simulink model "Modulator_CTDT"  (R2025b)
settings: Solver=ode4  StartTime=0.0  StopTime=0.5  FixedStep=Ts/10  MaxStep=1e-6  RelTol=1e-3
values from neighbouring files (symbols this model uses):
  Fs = 512e3    (= 512000)    [initialize_parameters_CTDT.m]
  Ts = 1/Fs    (= 1.953125e-06)    [initialize_parameters_CTDT.m]
undefined symbols (not defined in the file or in its folder): den, dspblkCoreblockFVToolHelper, gcbh, num
libraries: dspmlti4 x1
settings Model: Creator=anurag jaiswal  LastModifiedBy=divijsharma
settings DataIOCC: SaveOutput=off  SignalLogging=off  DSMLogging=off  SaveTime=off  ReturnWorkspaceOutputs=off

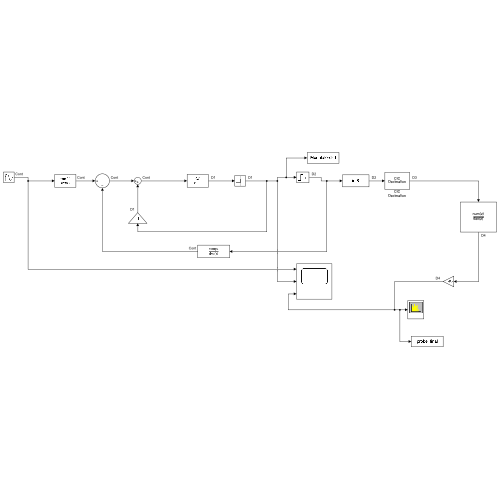
[thumbnail: Simulink's stored preview of the top-level diagram]
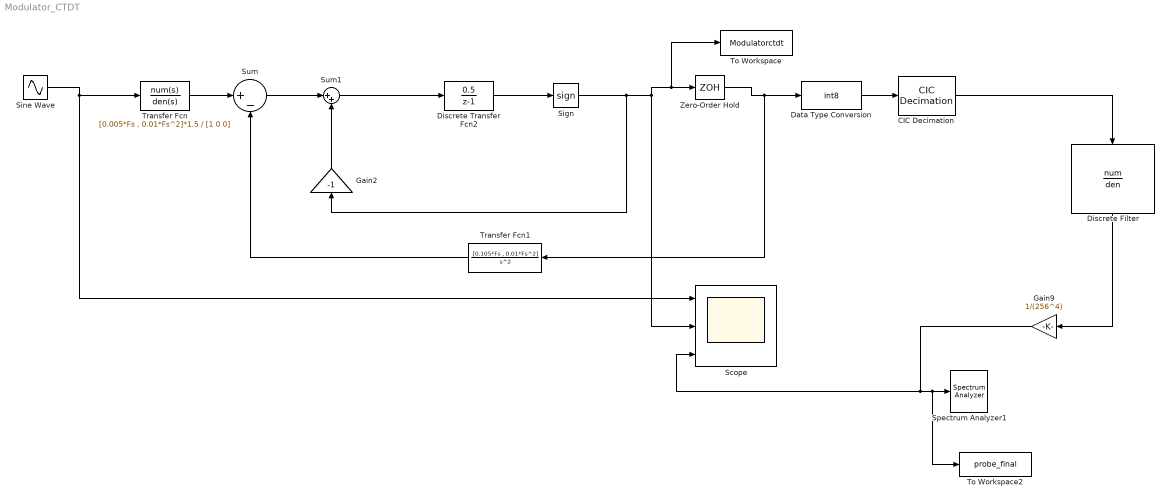
== system Modulator_CTDT ==
  CIC Decimation : dspmlti4/CIC Decimation  filtFrom=Dialog parameters  filtobj=CICDECIM  ftype=Decimator  R=256  M=1  N=5  filterInternals=Minimum section word lengths  BPS=[16 16 16 16]  FLPS=0  outputWordLength=32  outputFracLength=0  launchFVT=off  framing=Maintain input frame rate  RateOptions=Allow multirate processing
      settings: LibrarySourceBlock=|
      | dsphdlsupportfiltering/CIC
      | Decimation
  Data Type Conversion : DataTypeConversion  OutDataTypeStr=int8  SaturateOnIntegerOverflow=off  RndMeth=Floor
  Discrete Transfer Fcn2 : DiscreteTransferFcn  LoadFcn=dspblkCoreblockFVToolHelper(gcbh,'load');  Numerator=[0.5]  Denominator=[1 -1]
      settings: CopyFcn=dspblkCoreblockFVToolHelper(gcbh,'copy');  DeleteFcn=dspblkCoreblockFVToolHelper(gcbh,'close');  ModelCloseFcn=dspblkCoreblockFVToolHelper(gcbh,'close');  PreSaveFcn=dspblkCoreblockFVToolHelper(gcbh,'presave');  PostSaveFcn=dspblkCoreblockFVToolHelper(gcbh,'postsave');  CloseFcn=dspblkCoreblockFVToolHelper(gcbh,'close');
  Discrete Filter : DiscreteFilter  LoadFcn=dspblkCoreblockFVToolHelper(gcbh,'load');  Numerator=num  Denominator=den
      settings: CopyFcn=dspblkCoreblockFVToolHelper(gcbh,'copy');  DeleteFcn=dspblkCoreblockFVToolHelper(gcbh,'close');  ModelCloseFcn=dspblkCoreblockFVToolHelper(gcbh,'close');  PreSaveFcn=dspblkCoreblockFVToolHelper(gcbh,'presave');  PostSaveFcn=dspblkCoreblockFVToolHelper(gcbh,'postsave');  CloseFcn=dspblkCoreblockFVToolHelper(gcbh,'close');
  Gain2 : Gain  Gain=-1
  Gain9 : Gain  Gain=1/(256^4)
  Scope : Scope  NumInputPorts=3
      settings: ActiveDisplayYMinimum=-0.125  ActiveDisplayYMaximum=0.125
  Sign : Signum
  Sine Wave : Sin  Amplitude=0.1  Frequency=2*pi*100  SampleTime=0
  Spectrum Analyzer1 : SpectrumAnalyzer  WindowPosition=[-128.000000,1.000000,1536.000000,741.000000,]  Visible=on  ScopeFrameLocation=window  WindowInvariantSamplesPerUpdate=on  Span=4000  StartFrequency=-2000  StopFrequency=2000  YLimits=[-15.248 62.5405]  SelectedToolstripTab=spectrumAnalyzerToolstrip.channelMeasurementsTab
  Sum : Sum  Inputs=|+-
  Sum1 : Sum  Inputs=|++
  To Workspace : ToWorkspace  VariableName=Modulatorctdt  SampleTime=-1
  To Workspace2 : ToWorkspace  VariableName=probe_final  SampleTime=-1
      settings: Save2DSignal=2-D array (concatenate along first dimension)
  Transfer Fcn : TransferFcn  Numerator=[0.005*Fs , 0.01*Fs^2]*1.5  Denominator=[1 0 0]
  Transfer Fcn1 : TransferFcn  Numerator=[0.105*Fs , 0.01*Fs^2]  Denominator=[1 0 0]
  Zero-Order Hold : ZeroOrderHold  SampleTime=Ts
  wires:
  Sum/1 -> Sum1/1
  Sine Wave/1 -> Transfer Fcn/1, Scope/1
  Transfer Fcn/1 -> Sum/1
  Sum1/1 -> Discrete Transfer Fcn2/1
  Gain2/1 -> Sum1/2
  Transfer Fcn1/1 -> Sum/2
  Data Type Conversion/1 -> CIC Decimation/1
  Zero-Order Hold/1 -> Transfer Fcn1/1, Data Type Conversion/1
  Gain9/1 -> Scope/3, To Workspace2/1, Spectrum Analyzer1/1
  Discrete Transfer Fcn2/1 -> Sign/1
  Sign/1 -> Zero-Order Hold/1, To Workspace/1, Scope/2, Gain2/1
  Discrete Filter/1 -> Gain9/1
  CIC Decimation/1 -> Discrete Filter/1
